simulink model "Simscape_Drone_Model"  (R2025b)
settings: Solver=FixedStepAuto  StartTime=0.0  StopTime=10  RelTol=1e-6  EnableMultiTasking=on
undefined symbols (not defined in the file): Aero_On, Config, P, SimParams, SimscapeParams, X, Y, Z
libraries: sm_lib x89, nesl_utility x71, fl_lib x18, sdl_lib x8, slpidlib x4, batteryecm_lib x1
(part 4 of 5)

== system Simscape_Drone_Model/Drone Mechanical/Motor Holder 1 ==
  rho : Inport
  Motor Holder 1 : sm_lib/Body Elements/Cylindrical Solid  CylinderRadius=SimscapeParams.MotorRadius  CylinderRadiusUnits=m  CylinderLength=SimscapeParams.MotorHeight  CylinderLengthUnits=m  ExportEntireGeometry=off  InertiaType=CalculateFromGeometry  BasedOnType=Mass  Density=1000  DensityUnits=kg/m^3  Mass=SimscapeParams.MotorMass  MassUnits=kg  CenterOfMass=[0 0 0]  CenterOfMassUnits=m  MomentsOfInertia=[1 1 1]  MomentsOfInertiaUnits=kg*m^2  ProductsOfInertia=[0 0 0]  ProductsOfInertiaUnits=kg*m^2  GraphicType=FromGeometry  MarkerShape=Sphere  MarkerSize=10  GraphicVisPropType=SimpleVisualProperties  GraphicDiffuseColor=[0.898 1 0]  GraphicOpacity=1  GraphicSpecularColor=[0.5 0.5 0.5 1.0]  GraphicAmbientColor=[0.15 0.15 0.15 1.0]  GraphicEmissiveColor=[0.0 0.0 0.0 1.0]  GraphicShininess=75  DoExposeReferenceFrame=off  SerializedFrames=|
      | <Frames>
      | 
      |   <Frame>
      |     <Id>Frame1</Id>
      |     <Value>
      |       <Name>Top</Name>
      |       <Origin>
      |         <Source>GeometricFeature</Source>
      |         <FeatureName>bottom surface</FeatureName>
      |       </Origin>
      |       <PrimaryAxis>
      |         <DefinedDirection>+Z</DefinedDirection>
      |         <Source>ReferenceFrame</Source>
      |         <SourceDirection>+Z</SourceDirection>
      |         <FeatureName></FeatureName>
      |       </PrimaryAxis>
      |       <SecondaryAxis>
      |         <DefinedDirection>+X</DefinedDirection>
      |         <Source>ReferenceFrame</Source>
      |         <SourceDirection>+X</SourceDirection>
      |         <FeatureName></FeatureName>
      |       </SecondaryAxis>
      |     </Value>
      |   </Frame>
      | 
      |   <Frame>
      |     <Id>Frame2</Id>
      |     <Value>
      |       <Name>Side</Name>
      |       <Origin>
      |         <Source>GeometricFeature</Source>
      |         <FeatureName>side surface</FeatureName>
      |       </Origin>
      |       <PrimaryAxis>
      |         <DefinedDirection>+Z</DefinedDirection>
      |         <Source>ReferenceFrame</Source>
      |         <SourceDirection>+Z</SourceDirection>
      |         <FeatureName></FeatureName>
      |       </PrimaryAxis>
      |       <SecondaryAxis>
      |         <DefinedDirection>+X</DefinedDirection>
      |         <Source>ReferenceFrame</Source>
      |         <SourceDirection>-X</SourceDirection>
      |         <FeatureName></FeatureName>
      |       </SecondaryAxis>
      |     </Value>
      |   </Frame>
      | 
      | </Frames>
  Rigid Transform : sm_lib/Frames and Transforms/Rigid Transform  RotationMethod=ArbitraryAxis  FollAlignAxisA=+X  BaseAlignAxisA=+Y  FollAlignAxisB=+Y  BaseAlignAxisB=+Z  RotationStandardAxis=+Z  RotationAngle=SimscapeParams.MotorHolderRotationAngle  RotationAngleUnits=deg  RotationArbitraryAxis=SimscapeParams.MotorHolderRotationAxis1  RotationSequenceAxes=FollowerAxes  RotationSequence=YXY  RotationSequenceAngles=[0 90 0]  RotationSequenceAnglesUnits=deg  RotationMatrix=[1 0 0;0 1 0;0 0 1]  Quaternion=[1 0 0 0]  TranslationMethod=None  TranslationCartesianOffset=[0 0 0]  TranslationCartesianOffsetUnits=m  TranslationStandardAxis=+Z  TranslationStandardOffset=0  TranslationStandardOffsetUnits=m  TranslationROffset=0  TranslationROffsetUnits=m  TranslationThetaOffset=0  TranslationThetaOffsetUnits=deg  TranslationZOffset=0  TranslationZOffsetUnits=m
  Subsystem : Subsystem
  NED : PMIOPort  Side=Left
  Connection : PMIOPort  Port=2  Side=Left
  Side : PMIOPort  Port=3  Side=Left
  Propeller : PMIOPort  Port=4  Side=Right
  wires:
  rho/1 -> Subsystem/1(rho)
  connections:
  Rigid Transform/LConn1 -- Connection/RConn1
  Motor Holder 1/LConn1 -- Propeller/RConn1
  Rigid Transform/RConn1 -- Motor Holder 1/RConn1 -- Subsystem/RConn2 -- Subsystem/RConn1 -- Side/RConn1
  NED/RConn1 -- Subsystem/LConn1

== system Simscape_Drone_Model/Drone Mechanical/Motor Holder 2 ==
  rho : Inport
  Aero Dynamic Drag : Subsystem
  External Force and Torque : sm_lib/Forces and Torques/External Force and Torque  EnableForceX=off  EnableForceY=off  EnableForceZ=off  EnableForce=on  ForceResolutionFrame=AttachedFrame  EnableTorqueX=off  EnableTorqueY=off  EnableTorqueZ=off  EnableTorque=off  TorqueResolutionFrame=AttachedFrame
  Motor Holder 2 : sm_lib/Body Elements/Cylindrical Solid  CylinderRadius=SimscapeParams.MotorRadius  CylinderRadiusUnits=m  CylinderLength=SimscapeParams.MotorHeight  CylinderLengthUnits=m  ExportEntireGeometry=off  InertiaType=CalculateFromGeometry  BasedOnType=Mass  Density=1000  DensityUnits=kg/m^3  Mass=SimscapeParams.MotorMass  MassUnits=kg  CenterOfMass=[0 0 0]  CenterOfMassUnits=m  MomentsOfInertia=[1 1 1]  MomentsOfInertiaUnits=kg*m^2  ProductsOfInertia=[0 0 0]  ProductsOfInertiaUnits=kg*m^2  GraphicType=FromGeometry  MarkerShape=Sphere  MarkerSize=10  GraphicVisPropType=SimpleVisualProperties  GraphicDiffuseColor=[0.898 1 0]  GraphicOpacity=1  GraphicSpecularColor=[0.5 0.5 0.5 1.0]  GraphicAmbientColor=[0.15 0.15 0.15 1.0]  GraphicEmissiveColor=[0.0 0.0 0.0 1.0]  GraphicShininess=75  DoExposeReferenceFrame=off  SerializedFrames=|
      | <Frames>
      | 
      |   <Frame>
      |     <Id>Frame1</Id>
      |     <Value>
      |       <Name>Top</Name>
      |       <Origin>
      |         <Source>GeometricFeature</Source>
      |         <FeatureName>bottom surface</FeatureName>
      |       </Origin>
      |       <PrimaryAxis>
      |         <DefinedDirection>+Z</DefinedDirection>
      |         <Source>ReferenceFrame</Source>
      |         <SourceDirection>+Z</SourceDirection>
      |         <FeatureName></FeatureName>
      |       </PrimaryAxis>
      |       <SecondaryAxis>
      |         <DefinedDirection>+X</DefinedDirection>
      |         <Source>ReferenceFrame</Source>
      |         <SourceDirection>+X</SourceDirection>
      |         <FeatureName></FeatureName>
      |       </SecondaryAxis>
      |     </Value>
      |   </Frame>
      | 
      |   <Frame>
      |     <Id>Frame2</Id>
      |     <Value>
      |       <Name>Side</Name>
      |       <Origin>
      |         <Source>GeometricFeature</Source>
      |         <FeatureName>side surface</FeatureName>
      |       </Origin>
      |       <PrimaryAxis>
      |         <DefinedDirection>+Z</DefinedDirection>
      |         <Source>ReferenceFrame</Source>
      |         <SourceDirection>+Z</SourceDirection>
      |         <FeatureName></FeatureName>
      |       </PrimaryAxis>
      |       <SecondaryAxis>
      |         <DefinedDirection>+X</DefinedDirection>
      |         <Source>ReferenceFrame</Source>
      |         <SourceDirection>-X</SourceDirection>
      |         <FeatureName></FeatureName>
      |       </SecondaryAxis>
      |     </Value>
      |   </Frame>
      | 
      | </Frames>
  Rigid Transform : sm_lib/Frames and Transforms/Rigid Transform  RotationMethod=ArbitraryAxis  FollAlignAxisA=+X  BaseAlignAxisA=+Y  FollAlignAxisB=+Y  BaseAlignAxisB=+Z  RotationStandardAxis=+Z  RotationAngle=SimscapeParams.MotorHolderRotationAngle  RotationAngleUnits=deg  RotationArbitraryAxis=SimscapeParams.MotorHolderRotationAxis2  RotationSequenceAxes=BaseAxes  RotationSequence=XYX  RotationSequenceAngles=[0 90 0]  RotationSequenceAnglesUnits=deg  RotationMatrix=[1 0 0;0 1 0;0 0 1]  Quaternion=[1 0 0 0]  TranslationMethod=None  TranslationCartesianOffset=[0 0 0]  TranslationCartesianOffsetUnits=m  TranslationStandardAxis=+Z  TranslationStandardOffset=0  TranslationStandardOffsetUnits=m  TranslationROffset=0  TranslationROffsetUnits=m  TranslationThetaOffset=0  TranslationThetaOffsetUnits=deg  TranslationZOffset=0  TranslationZOffsetUnits=m
  Simulink-PS Converter : nesl_utility/Simulink-PS Converter  PhysicalDomain=network_engine_domain  SubClassName=ps_input  LeftPortType=input  RightPortType=output  PseudoPeriodic=off  Frequencies=[]  NoiseDistribution=none  NoiseParameters=[]  Unit=1  AffineConversion=off  FilteringAndDerivatives=provide  SimscapeFilterOrder=1  InputFilterTimeConstant=0.001  UdotUserProvided=0
  NED : PMIOPort  Side=Left
  Connection : PMIOPort  Port=2  Side=Left
  Side : PMIOPort  Port=3  Side=Left
  Propeller : PMIOPort  Port=4  Side=Right
  wires:
  Aero Dynamic Drag/1(F_drag) -> Simulink-PS Converter/1
  rho/1 -> Aero Dynamic Drag/1(rho)
  connections:
  External Force and Torque/LConn1 -- Simulink-PS Converter/RConn1
  Aero Dynamic Drag/LConn1 -- NED/RConn1
  Rigid Transform/LConn1 -- Connection/RConn1
  Side/RConn1 -- Rigid Transform/RConn1 -- External Force and Torque/RConn1 -- Aero Dynamic Drag/LConn2 -- Motor Holder 2/RConn1
  Motor Holder 2/LConn1 -- Propeller/RConn1

== system Simscape_Drone_Model/Drone Mechanical/Motor Holder 3 ==
  rho : Inport
  Aero Dynamic Drag : Subsystem
  External Force and Torque : sm_lib/Forces and Torques/External Force and Torque  EnableForceX=off  EnableForceY=off  EnableForceZ=off  EnableForce=on  ForceResolutionFrame=AttachedFrame  EnableTorqueX=off  EnableTorqueY=off  EnableTorqueZ=off  EnableTorque=off  TorqueResolutionFrame=AttachedFrame
  Motor Holder 3 : sm_lib/Body Elements/Cylindrical Solid  CylinderRadius=SimscapeParams.MotorRadius  CylinderRadiusUnits=m  CylinderLength=SimscapeParams.MotorHeight  CylinderLengthUnits=m  ExportEntireGeometry=off  InertiaType=CalculateFromGeometry  BasedOnType=Mass  Density=1000  DensityUnits=kg/m^3  Mass=SimscapeParams.MotorMass  MassUnits=kg  CenterOfMass=[0 0 0]  CenterOfMassUnits=m  MomentsOfInertia=[1 1 1]  MomentsOfInertiaUnits=kg*m^2  ProductsOfInertia=[0 0 0]  ProductsOfInertiaUnits=kg*m^2  GraphicType=FromGeometry  MarkerShape=Sphere  MarkerSize=10  GraphicVisPropType=SimpleVisualProperties  GraphicDiffuseColor=[0.898 1 0]  GraphicOpacity=1  GraphicSpecularColor=[0.5 0.5 0.5 1.0]  GraphicAmbientColor=[0.15 0.15 0.15 1.0]  GraphicEmissiveColor=[0.0 0.0 0.0 1.0]  GraphicShininess=75  DoExposeReferenceFrame=off  SerializedFrames=|
      | <Frames>
      | 
      |   <Frame>
      |     <Id>Frame1</Id>
      |     <Value>
      |       <Name>Top</Name>
      |       <Origin>
      |         <Source>GeometricFeature</Source>
      |         <FeatureName>bottom surface</FeatureName>
      |       </Origin>
      |       <PrimaryAxis>
      |         <DefinedDirection>+Z</DefinedDirection>
      |         <Source>ReferenceFrame</Source>
      |         <SourceDirection>+Z</SourceDirection>
      |         <FeatureName></FeatureName>
      |       </PrimaryAxis>
      |       <SecondaryAxis>
      |         <DefinedDirection>+X</DefinedDirection>
      |         <Source>ReferenceFrame</Source>
      |         <SourceDirection>+X</SourceDirection>
      |         <FeatureName></FeatureName>
      |       </SecondaryAxis>
      |     </Value>
      |   </Frame>
      | 
      |   <Frame>
      |     <Id>Frame2</Id>
      |     <Value>
      |       <Name>Side</Name>
      |       <Origin>
      |         <Source>GeometricFeature</Source>
      |         <FeatureName>side surface</FeatureName>
      |       </Origin>
      |       <PrimaryAxis>
      |         <DefinedDirection>+Z</DefinedDirection>
      |         <Source>ReferenceFrame</Source>
      |         <SourceDirection>+Z</SourceDirection>
      |         <FeatureName></FeatureName>
      |       </PrimaryAxis>
      |       <SecondaryAxis>
      |         <DefinedDirection>+X</DefinedDirection>
      |         <Source>ReferenceFrame</Source>
      |         <SourceDirection>-X</SourceDirection>
      |         <FeatureName></FeatureName>
      |       </SecondaryAxis>
      |     </Value>
      |   </Frame>
      | 
      | </Frames>
  Rigid Transform : sm_lib/Frames and Transforms/Rigid Transform  RotationMethod=ArbitraryAxis  FollAlignAxisA=+X  BaseAlignAxisA=+Y  FollAlignAxisB=+Y  BaseAlignAxisB=+Z  RotationStandardAxis=+Z  RotationAngle=SimscapeParams.MotorHolderRotationAngle  RotationAngleUnits=deg  RotationArbitraryAxis=SimscapeParams.MotorHolderRotationAxis3  RotationSequenceAxes=FollowerAxes  RotationSequence=YXY  RotationSequenceAngles=[0 90 0]  RotationSequenceAnglesUnits=deg  RotationMatrix=[1 0 0;0 1 0;0 0 1]  Quaternion=[1 0 0 0]  TranslationMethod=None  TranslationCartesianOffset=[0 0 0]  TranslationCartesianOffsetUnits=m  TranslationStandardAxis=+Z  TranslationStandardOffset=0  TranslationStandardOffsetUnits=m  TranslationROffset=0  TranslationROffsetUnits=m  TranslationThetaOffset=0  TranslationThetaOffsetUnits=deg  TranslationZOffset=0  TranslationZOffsetUnits=m
  Simulink-PS Converter : nesl_utility/Simulink-PS Converter  PhysicalDomain=network_engine_domain  SubClassName=ps_input  LeftPortType=input  RightPortType=output  PseudoPeriodic=off  Frequencies=[]  NoiseDistribution=none  NoiseParameters=[]  Unit=1  AffineConversion=off  FilteringAndDerivatives=provide  SimscapeFilterOrder=1  InputFilterTimeConstant=0.001  UdotUserProvided=0
  NED : PMIOPort  Side=Left
  Connection : PMIOPort  Port=2  Side=Left
  Propeller : PMIOPort  Port=3  Side=Right
  Side : PMIOPort  Port=4  Side=Right
  wires:
  rho/1 -> Aero Dynamic Drag/1(rho)
  Aero Dynamic Drag/1(F_drag) -> Simulink-PS Converter/1
  connections:
  Aero Dynamic Drag/LConn1 -- NED/RConn1
  External Force and Torque/LConn1 -- Simulink-PS Converter/RConn1
  Rigid Transform/LConn1 -- Connection/RConn1
  Rigid Transform/RConn1 -- Motor Holder 3/RConn1 -- Side/RConn1 -- Aero Dynamic Drag/LConn2 -- External Force and Torque/RConn1
  Propeller/RConn1 -- Motor Holder 3/LConn1

== system Simscape_Drone_Model/Drone Mechanical/Motor Holder 4 ==
  rho : Inport
  Aero Dynamic Drag : Subsystem
  External Force and Torque : sm_lib/Forces and Torques/External Force and Torque  EnableForceX=off  EnableForceY=off  EnableForceZ=off  EnableForce=on  ForceResolutionFrame=AttachedFrame  EnableTorqueX=off  EnableTorqueY=off  EnableTorqueZ=off  EnableTorque=off  TorqueResolutionFrame=AttachedFrame
  Motor Holder 4 : sm_lib/Body Elements/Cylindrical Solid  CylinderRadius=SimscapeParams.MotorRadius  CylinderRadiusUnits=m  CylinderLength=SimscapeParams.MotorHeight  CylinderLengthUnits=m  ExportEntireGeometry=off  InertiaType=CalculateFromGeometry  BasedOnType=Mass  Density=1000  DensityUnits=kg/m^3  Mass=SimscapeParams.MotorMass  MassUnits=kg  CenterOfMass=[0 0 0]  CenterOfMassUnits=m  MomentsOfInertia=[1 1 1]  MomentsOfInertiaUnits=kg*m^2  ProductsOfInertia=[0 0 0]  ProductsOfInertiaUnits=kg*m^2  GraphicType=FromGeometry  MarkerShape=Sphere  MarkerSize=10  GraphicVisPropType=SimpleVisualProperties  GraphicDiffuseColor=[0.898 1 0]  GraphicOpacity=1  GraphicSpecularColor=[0.5 0.5 0.5 1.0]  GraphicAmbientColor=[0.15 0.15 0.15 1.0]  GraphicEmissiveColor=[0.0 0.0 0.0 1.0]  GraphicShininess=75  DoExposeReferenceFrame=off  SerializedFrames=|
      | <Frames>
      | 
      |   <Frame>
      |     <Id>Frame1</Id>
      |     <Value>
      |       <Name>Top</Name>
      |       <Origin>
      |         <Source>GeometricFeature</Source>
      |         <FeatureName>bottom surface</FeatureName>
      |       </Origin>
      |       <PrimaryAxis>
      |         <DefinedDirection>+Z</DefinedDirection>
      |         <Source>ReferenceFrame</Source>
      |         <SourceDirection>+Z</SourceDirection>
      |         <FeatureName></FeatureName>
      |       </PrimaryAxis>
      |       <SecondaryAxis>
      |         <DefinedDirection>+X</DefinedDirection>
      |         <Source>ReferenceFrame</Source>
      |         <SourceDirection>+X</SourceDirection>
      |         <FeatureName></FeatureName>
      |       </SecondaryAxis>
      |     </Value>
      |   </Frame>
      | 
      |   <Frame>
      |     <Id>Frame2</Id>
      |     <Value>
      |       <Name>Side</Name>
      |       <Origin>
      |         <Source>GeometricFeature</Source>
      |         <FeatureName>side surface</FeatureName>
      |       </Origin>
      |       <PrimaryAxis>
      |         <DefinedDirection>+Z</DefinedDirection>
      |         <Source>ReferenceFrame</Source>
      |         <SourceDirection>+Z</SourceDirection>
      |         <FeatureName></FeatureName>
      |       </PrimaryAxis>
      |       <SecondaryAxis>
      |         <DefinedDirection>+X</DefinedDirection>
      |         <Source>ReferenceFrame</Source>
      |         <SourceDirection>-X</SourceDirection>
      |         <FeatureName></FeatureName>
      |       </SecondaryAxis>
      |     </Value>
      |   </Frame>
      | 
      | </Frames>
  Rigid Transform : sm_lib/Frames and Transforms/Rigid Transform  RotationMethod=ArbitraryAxis  FollAlignAxisA=+X  BaseAlignAxisA=+Y  FollAlignAxisB=+Y  BaseAlignAxisB=+Z  RotationStandardAxis=+Z  RotationAngle=SimscapeParams.MotorHolderRotationAngle  RotationAngleUnits=deg  RotationArbitraryAxis=SimscapeParams.MotorHolderRotationAxis4  RotationSequenceAxes=FollowerAxes  RotationSequence=YXY  RotationSequenceAngles=[0 90 0]  RotationSequenceAnglesUnits=deg  RotationMatrix=[1 0 0;0 1 0;0 0 1]  Quaternion=[1 0 0 0]  TranslationMethod=None  TranslationCartesianOffset=[0 0 0]  TranslationCartesianOffsetUnits=m  TranslationStandardAxis=+Z  TranslationStandardOffset=0  TranslationStandardOffsetUnits=m  TranslationROffset=0  TranslationROffsetUnits=m  TranslationThetaOffset=0  TranslationThetaOffsetUnits=deg  TranslationZOffset=0  TranslationZOffsetUnits=m
  Simulink-PS Converter : nesl_utility/Simulink-PS Converter  PhysicalDomain=network_engine_domain  SubClassName=ps_input  LeftPortType=input  RightPortType=output  PseudoPeriodic=off  Frequencies=[]  NoiseDistribution=none  NoiseParameters=[]  Unit=1  AffineConversion=off  FilteringAndDerivatives=provide  SimscapeFilterOrder=1  InputFilterTimeConstant=0.001  UdotUserProvided=0
  NED : PMIOPort  Side=Left
  Connection : PMIOPort  Port=2  Side=Left
  Propeller : PMIOPort  Port=3  Side=Right
  Side : PMIOPort  Port=4  Side=Right
  wires:
  rho/1 -> Aero Dynamic Drag/1(rho)
  Aero Dynamic Drag/1(F_drag) -> Simulink-PS Converter/1
  connections:
  Aero Dynamic Drag/LConn1 -- NED/RConn1
  External Force and Torque/LConn1 -- Simulink-PS Converter/RConn1
  Rigid Transform/LConn1 -- Connection/RConn1
  Rigid Transform/RConn1 -- Side/RConn1 -- Motor Holder 4/RConn1 -- External Force and Torque/RConn1 -- Aero Dynamic Drag/LConn2
  Motor Holder 4/LConn1 -- Propeller/RConn1

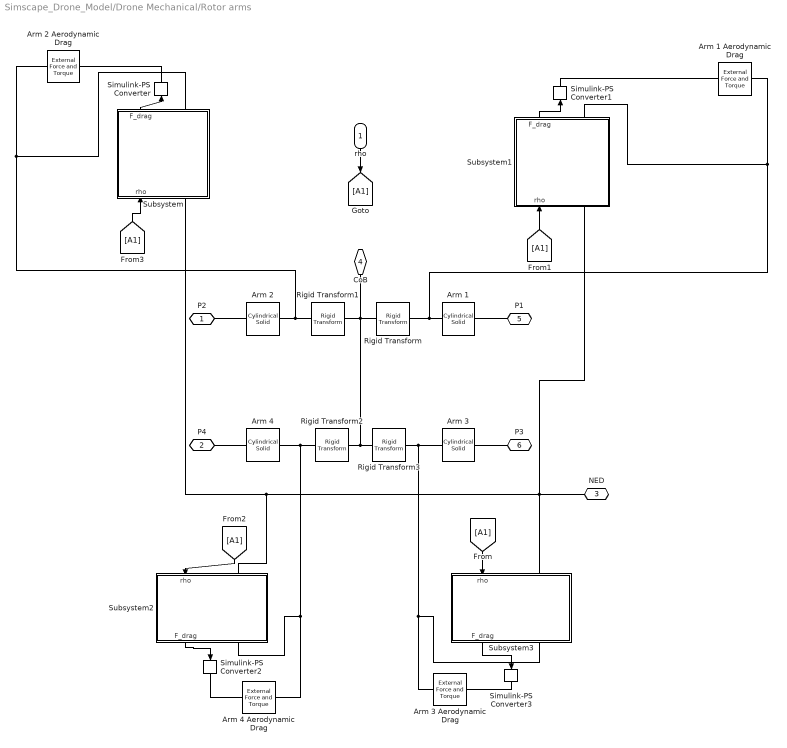
== system Simscape_Drone_Model/Drone Mechanical/Rotor arms ==
  rho : Inport
  Arm 1 : sm_lib/Body Elements/Cylindrical Solid  CylinderRadius=SimscapeParams.ArmRadius  CylinderRadiusUnits=m  CylinderLength=SimscapeParams.ArmLength  CylinderLengthUnits=m  ExportEntireGeometry=off  InertiaType=CalculateFromGeometry  BasedOnType=Mass  Density=1000  DensityUnits=kg/m^3  Mass=SimscapeParams.ArmMass  MassUnits=kg  CenterOfMass=[0 0 0]  CenterOfMassUnits=m  MomentsOfInertia=[1 1 1]  MomentsOfInertiaUnits=kg*m^2  ProductsOfInertia=[0 0 0]  ProductsOfInertiaUnits=kg*m^2  GraphicType=FromGeometry  MarkerShape=Sphere  MarkerSize=10  GraphicVisPropType=SimpleVisualProperties  GraphicDiffuseColor=[0 0.702 1]  GraphicOpacity=1  GraphicSpecularColor=[0.5 0.5 0.5 1.0]  GraphicAmbientColor=[0.15 0.15 0.15 1.0]  GraphicEmissiveColor=[0.0 0.0 0.0 1.0]  GraphicShininess=75  DoExposeReferenceFrame=on  SerializedFrames=|
      | <Frames>
      | 
      |   <Frame>
      |     <Id>Frame1</Id>
      |     <Value>
      |       <Name>F2</Name>
      |       <Origin>
      |         <Source>GeometricFeature</Source>
      |         <FeatureName>top surface</FeatureName>
      |       </Origin>
      |       <PrimaryAxis>
      |         <DefinedDirection>+Z</DefinedDirection>
      |         <Source>ReferenceFrame</Source>
      |         <SourceDirection>+Z</SourceDirection>
      |         <FeatureName></FeatureName>
      |       </PrimaryAxis>
      |       <SecondaryAxis>
      |         <DefinedDirection>+X</DefinedDirection>
      |         <Source>ReferenceFrame</Source>
      |         <SourceDirection>+X</SourceDirection>
      |         <FeatureName></FeatureName>
      |       </SecondaryAxis>
      |     </Value>
      |   </Frame>
      | 
      | </Frames>
  Arm 1 Aerodynamic Drag : sm_lib/Forces and Torques/External Force and Torque  EnableForceX=off  EnableForceY=off  EnableForceZ=off  EnableForce=on  ForceResolutionFrame=AttachedFrame  EnableTorqueX=off  EnableTorqueY=off  EnableTorqueZ=off  EnableTorque=off  TorqueResolutionFrame=AttachedFrame
  Arm 2 : sm_lib/Body Elements/Cylindrical Solid  CylinderRadius=SimscapeParams.ArmRadius  CylinderRadiusUnits=m  CylinderLength=SimscapeParams.ArmLength  CylinderLengthUnits=m  ExportEntireGeometry=off  InertiaType=CalculateFromGeometry  BasedOnType=Mass  Density=1000  DensityUnits=kg/m^3  Mass=SimscapeParams.ArmMass  MassUnits=kg  CenterOfMass=[0 0 0]  CenterOfMassUnits=m  MomentsOfInertia=[1 1 1]  MomentsOfInertiaUnits=kg*m^2  ProductsOfInertia=[0 0 0]  ProductsOfInertiaUnits=kg*m^2  GraphicType=FromGeometry  MarkerShape=Sphere  MarkerSize=10  GraphicVisPropType=SimpleVisualProperties  GraphicDiffuseColor=[0 0.702 1]  GraphicOpacity=1  GraphicSpecularColor=[0.5 0.5 0.5 1.0]  GraphicAmbientColor=[0.15 0.15 0.15 1.0]  GraphicEmissiveColor=[0.0 0.0 0.0 1.0]  GraphicShininess=75  DoExposeReferenceFrame=on  SerializedFrames=|
      | <Frames>
      | 
      |   <Frame>
      |     <Id>Frame1</Id>
      |     <Value>
      |       <Name>F2</Name>
      |       <Origin>
      |         <Source>GeometricFeature</Source>
      |         <FeatureName>top surface</FeatureName>
      |       </Origin>
      |       <PrimaryAxis>
      |         <DefinedDirection>+Z</DefinedDirection>
      |         <Source>ReferenceFrame</Source>
      |         <SourceDirection>+Z</SourceDirection>
      |         <FeatureName></FeatureName>
      |       </PrimaryAxis>
      |       <SecondaryAxis>
      |         <DefinedDirection>+X</DefinedDirection>
      |         <Source>ReferenceFrame</Source>
      |         <SourceDirection>+X</SourceDirection>
      |         <FeatureName></FeatureName>
      |       </SecondaryAxis>
      |     </Value>
      |   </Frame>
      | 
      | </Frames>
  Arm 2 Aerodynamic Drag : sm_lib/Forces and Torques/External Force and Torque  EnableForceX=off  EnableForceY=off  EnableForceZ=off  EnableForce=on  ForceResolutionFrame=AttachedFrame  EnableTorqueX=off  EnableTorqueY=off  EnableTorqueZ=off  EnableTorque=off  TorqueResolutionFrame=AttachedFrame
  Arm 3 : sm_lib/Body Elements/Cylindrical Solid  CylinderRadius=SimscapeParams.ArmRadius  CylinderRadiusUnits=m  CylinderLength=SimscapeParams.ArmLength  CylinderLengthUnits=m  ExportEntireGeometry=off  InertiaType=CalculateFromGeometry  BasedOnType=Mass  Density=1000  DensityUnits=kg/m^3  Mass=SimscapeParams.ArmMass  MassUnits=kg  CenterOfMass=[0 0 0]  CenterOfMassUnits=m  MomentsOfInertia=[1 1 1]  MomentsOfInertiaUnits=kg*m^2  ProductsOfInertia=[0 0 0]  ProductsOfInertiaUnits=kg*m^2  GraphicType=FromGeometry  MarkerShape=Sphere  MarkerSize=10  GraphicVisPropType=SimpleVisualProperties  GraphicDiffuseColor=[0 0.702 1]  GraphicOpacity=1  GraphicSpecularColor=[0.5 0.5 0.5 1.0]  GraphicAmbientColor=[0.15 0.15 0.15 1.0]  GraphicEmissiveColor=[0.0 0.0 0.0 1.0]  GraphicShininess=75  DoExposeReferenceFrame=on  SerializedFrames=|
      | <Frames>
      | 
      |   <Frame>
      |     <Id>Frame1</Id>
      |     <Value>
      |       <Name>F2</Name>
      |       <Origin>
      |         <Source>GeometricFeature</Source>
      |         <FeatureName>top surface</FeatureName>
      |       </Origin>
      |       <PrimaryAxis>
      |         <DefinedDirection>+Z</DefinedDirection>
      |         <Source>ReferenceFrame</Source>
      |         <SourceDirection>+Z</SourceDirection>
      |         <FeatureName></FeatureName>
      |       </PrimaryAxis>
      |       <SecondaryAxis>
      |         <DefinedDirection>+X</DefinedDirection>
      |         <Source>ReferenceFrame</Source>
      |         <SourceDirection>+X</SourceDirection>
      |         <FeatureName></FeatureName>
      |       </SecondaryAxis>
      |     </Value>
      |   </Frame>
      | 
      | </Frames>
  Arm 3 Aerodynamic Drag : sm_lib/Forces and Torques/External Force and Torque  EnableForceX=off  EnableForceY=off  EnableForceZ=off  EnableForce=on  ForceResolutionFrame=AttachedFrame  EnableTorqueX=off  EnableTorqueY=off  EnableTorqueZ=off  EnableTorque=off  TorqueResolutionFrame=AttachedFrame
  Arm 4 : sm_lib/Body Elements/Cylindrical Solid  CylinderRadius=SimscapeParams.ArmRadius  CylinderRadiusUnits=m  CylinderLength=SimscapeParams.ArmLength  CylinderLengthUnits=m  ExportEntireGeometry=off  InertiaType=CalculateFromGeometry  BasedOnType=Mass  Density=1000  DensityUnits=kg/m^3  Mass=SimscapeParams.ArmMass  MassUnits=kg  CenterOfMass=[0 0 0]  CenterOfMassUnits=m  MomentsOfInertia=[1 1 1]  MomentsOfInertiaUnits=kg*m^2  ProductsOfInertia=[0 0 0]  ProductsOfInertiaUnits=kg*m^2  GraphicType=FromGeometry  MarkerShape=Sphere  MarkerSize=10  GraphicVisPropType=SimpleVisualProperties  GraphicDiffuseColor=[0 0.702 1]  GraphicOpacity=1  GraphicSpecularColor=[0.5 0.5 0.5 1.0]  GraphicAmbientColor=[0.15 0.15 0.15 1.0]  GraphicEmissiveColor=[0.0 0.0 0.0 1.0]  GraphicShininess=75  DoExposeReferenceFrame=on  SerializedFrames=|
      | <Frames>
      | 
      |   <Frame>
      |     <Id>Frame1</Id>
      |     <Value>
      |       <Name>F2</Name>
      |       <Origin>
      |         <Source>GeometricFeature</Source>
      |         <FeatureName>top surface</FeatureName>
      |       </Origin>
      |       <PrimaryAxis>
      |         <DefinedDirection>+Z</DefinedDirection>
      |         <Source>ReferenceFrame</Source>
      |         <SourceDirection>+Z</SourceDirection>
      |         <FeatureName></FeatureName>
      |       </PrimaryAxis>
      |       <SecondaryAxis>
      |         <DefinedDirection>+X</DefinedDirection>
      |         <Source>ReferenceFrame</Source>
      |         <SourceDirection>+X</SourceDirection>
      |         <FeatureName></FeatureName>
      |       </SecondaryAxis>
      |     </Value>
      |   </Frame>
      | 
      | </Frames>
  Arm 4 Aerodynamic Drag : sm_lib/Forces and Torques/External Force and Torque  EnableForceX=off  EnableForceY=off  EnableForceZ=off  EnableForce=on  ForceResolutionFrame=AttachedFrame  EnableTorqueX=off  EnableTorqueY=off  EnableTorqueZ=off  EnableTorque=off  TorqueResolutionFrame=AttachedFrame
  Rigid Transform : sm_lib/Frames and Transforms/Rigid Transform  RotationMethod=ArbitraryAxis  FollAlignAxisA=+X  BaseAlignAxisA=+Y  FollAlignAxisB=+Y  BaseAlignAxisB=+Z  RotationStandardAxis=+Z  RotationAngle=SimscapeParams.ArmRotationAngle  RotationAngleUnits=deg  RotationArbitraryAxis=SimscapeParams.ArmRotationAxis1  RotationSequenceAxes=FollowerAxes  RotationSequence=XYZ  RotationSequenceAngles=P.Arm.RotationAngle.*P.Arm.RotationAxis1  RotationSequenceAnglesUnits=deg  RotationMatrix=[1 0 0;0 1 0;0 0 1]  Quaternion=[1 0 0 0]  TranslationMethod=Cartesian  TranslationCartesianOffset=SimscapeParams.ArmPosition1  TranslationCartesianOffsetUnits=m  TranslationStandardAxis=+Z  TranslationStandardOffset=0  TranslationStandardOffsetUnits=m  TranslationROffset=0  TranslationROffsetUnits=m  TranslationThetaOffset=0  TranslationThetaOffsetUnits=deg  TranslationZOffset=0  TranslationZOffsetUnits=m
  Rigid Transform1 : sm_lib/Frames and Transforms/Rigid Transform  RotationMethod=ArbitraryAxis  FollAlignAxisA=+X  BaseAlignAxisA=+Y  FollAlignAxisB=+Y  BaseAlignAxisB=+Z  RotationStandardAxis=+Z  RotationAngle=SimscapeParams.ArmRotationAngle  RotationAngleUnits=deg  RotationArbitraryAxis=SimscapeParams.ArmRotationAxis2  RotationSequenceAxes=FollowerAxes  RotationSequence=XYZ  RotationSequenceAngles=[-90 -45 0]  RotationSequenceAnglesUnits=deg  RotationMatrix=[1 0 0;0 1 0;0 0 1]  Quaternion=[1 0 0 0]  TranslationMethod=Cartesian  TranslationCartesianOffset=SimscapeParams.ArmPosition2  TranslationCartesianOffsetUnits=m  TranslationStandardAxis=+Z  TranslationStandardOffset=0  TranslationStandardOffsetUnits=m  TranslationROffset=0  TranslationROffsetUnits=m  TranslationThetaOffset=0  TranslationThetaOffsetUnits=deg  TranslationZOffset=0  TranslationZOffsetUnits=m
  Rigid Transform2 : sm_lib/Frames and Transforms/Rigid Transform  RotationMethod=ArbitraryAxis  FollAlignAxisA=+X  BaseAlignAxisA=+Y  FollAlignAxisB=+Y  BaseAlignAxisB=+Z  RotationStandardAxis=+Z  RotationAngle=SimscapeParams.ArmRotationAngle  RotationAngleUnits=deg  RotationArbitraryAxis=SimscapeParams.ArmRotationAxis4  RotationSequenceAxes=FollowerAxes  RotationSequence=XYZ  RotationSequenceAngles=[-90 -45 0]  RotationSequenceAnglesUnits=deg  RotationMatrix=[1 0 0;0 1 0;0 0 1]  Quaternion=[1 0 0 0]  TranslationMethod=Cartesian  TranslationCartesianOffset=SimscapeParams.ArmPosition4  TranslationCartesianOffsetUnits=m  TranslationStandardAxis=+Z  TranslationStandardOffset=0  TranslationStandardOffsetUnits=m  TranslationROffset=0  TranslationROffsetUnits=m  TranslationThetaOffset=0  TranslationThetaOffsetUnits=deg  TranslationZOffset=0  TranslationZOffsetUnits=m
  Rigid Transform3 : sm_lib/Frames and Transforms/Rigid Transform  RotationMethod=ArbitraryAxis  FollAlignAxisA=+X  BaseAlignAxisA=+Y  FollAlignAxisB=+Y  BaseAlignAxisB=+Z  RotationStandardAxis=+Z  RotationAngle=SimscapeParams.ArmRotationAngle  RotationAngleUnits=deg  RotationArbitraryAxis=SimscapeParams.ArmRotationAxis3  RotationSequenceAxes=FollowerAxes  RotationSequence=XYZ  RotationSequenceAngles=[-90 -45 0]  RotationSequenceAnglesUnits=deg  RotationMatrix=[1 0 0;0 1 0;0 0 1]  Quaternion=[1 0 0 0]  TranslationMethod=Cartesian  TranslationCartesianOffset=SimscapeParams.ArmPosition3  TranslationCartesianOffsetUnits=m  TranslationStandardAxis=+Z  TranslationStandardOffset=0  TranslationStandardOffsetUnits=m  TranslationROffset=0  TranslationROffsetUnits=m  TranslationThetaOffset=0  TranslationThetaOffsetUnits=deg  TranslationZOffset=0  TranslationZOffsetUnits=m
  Simulink-PS Converter{,1..3} (4 alike) : nesl_utility/Simulink-PS Converter  PhysicalDomain=network_engine_domain  SubClassName=ps_input  LeftPortType=input  RightPortType=output  PseudoPeriodic=off  Frequencies=[]  NoiseDistribution=none  NoiseParameters=[]  Unit=1  AffineConversion=off  FilteringAndDerivatives=provide  SimscapeFilterOrder=1  InputFilterTimeConstant=0.001  UdotUserProvided=0
  Subsystem : Subsystem
  Subsystem1 : Subsystem
  Subsystem2 : Subsystem
  Subsystem3 : Subsystem
  P2 : PMIOPort  Side=Left
  P4 : PMIOPort  Port=2  Side=Left
  NED : PMIOPort  Port=3  Side=Left
  CoB : PMIOPort  Port=4  Side=Left
  P1 : PMIOPort  Port=5  Side=Right
  P3 : PMIOPort  Port=6  Side=Right
  wires:
  rho/1 -> [A1]
  [A1] -> Subsystem/1(rho)
  Subsystem/1(F_drag) -> Simulink-PS Converter/1
  [A1] -> Subsystem1/1(rho)
  Subsystem1/1(F_drag) -> Simulink-PS Converter1/1
  [A1] -> Subsystem2/1(rho)
  Subsystem2/1(F_drag) -> Simulink-PS Converter2/1
  [A1] -> Subsystem3/1(rho)
  Subsystem3/1(F_drag) -> Simulink-PS Converter3/1
  connections:
  Arm 3 Aerodynamic Drag/LConn1 -- Simulink-PS Converter3/RConn1
  Arm 4 Aerodynamic Drag/LConn1 -- Simulink-PS Converter2/RConn1
  P2/RConn1 -- Arm 2/LConn1
  Arm 4/LConn1 -- P4/RConn1
  Arm 3/LConn1 -- P3/RConn1
  Arm 1/LConn1 -- P1/RConn1
  Rigid Transform3/RConn1 -- Arm 3/RConn1 -- Subsystem3/RConn1 -- Arm 3 Aerodynamic Drag/RConn1
  Arm 1 Aerodynamic Drag/LConn1 -- Simulink-PS Converter1/RConn1
  Arm 2 Aerodynamic Drag/LConn1 -- Simulink-PS Converter/RConn1
  Arm 2/RConn1 -- Rigid Transform1/RConn1 -- Subsystem/RConn1 -- Arm 2 Aerodynamic Drag/RConn1
  Arm 1/RConn1 -- Rigid Transform/RConn1 -- Subsystem1/RConn1 -- Arm 1 Aerodynamic Drag/RConn1
  Rigid Transform1/LConn1 -- CoB/RConn1 -- Rigid Transform2/LConn1 -- Rigid Transform3/LConn1 -- Rigid Transform/LConn1
  Subsystem3/LConn1 -- Subsystem1/LConn1 -- NED/RConn1 -- Subsystem/LConn1 -- Subsystem2/LConn1
  Rigid Transform2/RConn1 -- Arm 4/RConn1 -- Arm 4 Aerodynamic Drag/RConn1 -- Subsystem2/RConn1

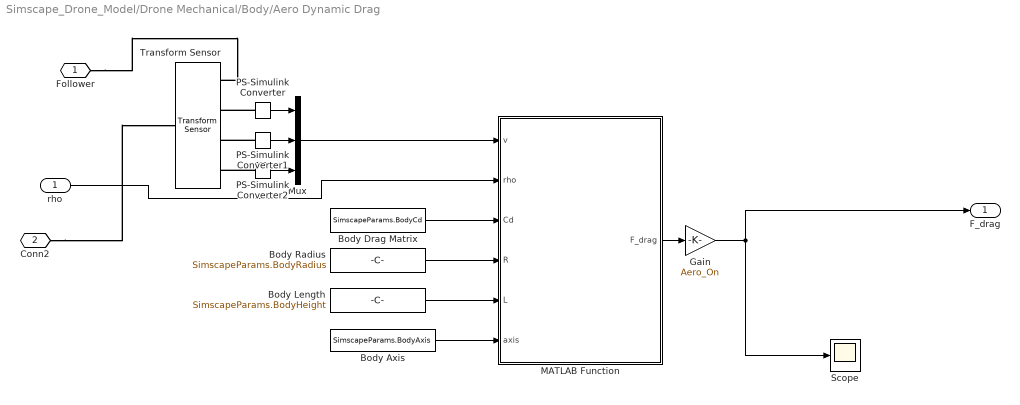
== system Simscape_Drone_Model/Drone Mechanical/Body/Aero Dynamic Drag ==
  rho : Inport
  Body Axis : Constant  Value=SimscapeParams.BodyAxis
  Body Drag Matrix : Constant  Value=SimscapeParams.BodyCd
  Body Length : Constant  Value=SimscapeParams.BodyHeight
  Body Radius : Constant  Value=SimscapeParams.BodyRadius
  Gain : Gain  Gain=Aero_On
  MATLAB Function : MATLAB Function  TreatAsAtomicUnit=on
  Mux : Mux  Inputs=3
  PS-Simulink Converter : nesl_utility/PS-Simulink Converter  PhysicalDomain=network_engine_domain  SubClassName=ps_output  LeftPortType=input  RightPortType=output  PseudoPeriodic=off  Frequencies=[]  VectorFormat=inherit  Unit=inherit  AffineConversion=off
  PS-Simulink Converter1 : nesl_utility/PS-Simulink Converter  PhysicalDomain=network_engine_domain  SubClassName=ps_output  LeftPortType=input  RightPortType=output  PseudoPeriodic=off  Frequencies=[]  VectorFormat=inherit  Unit=inherit  AffineConversion=off
  PS-Simulink Converter2 : nesl_utility/PS-Simulink Converter  PhysicalDomain=network_engine_domain  SubClassName=ps_output  LeftPortType=input  RightPortType=output  PseudoPeriodic=off  Frequencies=[]  VectorFormat=inherit  Unit=inherit  AffineConversion=off
  Scope : Scope
      settings: ActiveDisplayYMinimum=-1  ActiveDisplayYMaximum=1  DataLoggingVariableName=ScopeData4
  Transform Sensor : sm_lib/Frames and Transforms/Transform Sensor  MeasurementFrame=NonRotatingFollower  RotationSequence=XYZ  SenseAngle=off  SenseAxis=off  SenseQ=off  SenseR=off  SenseRotationSequence=off  SenseOmegaX=off  SenseOmegaY=off  SenseOmegaZ=off  SenseOmega=off  SenseQDot=off  SenseRDot=off  SenseRotationSequenceDot=off  SenseAlphaX=off  SenseAlphaY=off  SenseAlphaZ=off  SenseAlpha=off  SenseQDDot=off  SenseRDDot=off  SenseX=off  SenseY=off  SenseZ=off  SenseXYZ=off  SenseRad=off  SenseAzim=off  SenseDist=off  SenseInc=off  SenseXDot=on  SenseYDot=on  SenseZDot=on  SenseXYZDot=off  SenseRadDot=off  SenseAzimDot=off  SenseDistDot=off  SenseIncDot=off  SenseXDDot=off  SenseYDDot=off  SenseZDDot=off  SenseXYZDDot=off  SenseRadDDot=off  SenseAzimDDot=off  SenseDistDDot=off  SenseIncDDot=off
  Follower : PMIOPort  Side=Right
  Conn2 : PMIOPort  Port=2  Side=Left
  F_drag : Outport
  wires:
  Body Axis/1 -> MATLAB Function/6(axis)
  Body Drag Matrix/1 -> MATLAB Function/3(Cd)
  PS-Simulink Converter/1 -> Mux/1
  PS-Simulink Converter1/1 -> Mux/2
  Body Radius/1 -> MATLAB Function/4(R)
  Body Length/1 -> MATLAB Function/5(L)
  MATLAB Function/1(F_drag) -> Gain/1
  rho/1 -> MATLAB Function/2(rho)
  PS-Simulink Converter2/1 -> Mux/3
  Mux/1 -> MATLAB Function/1(v)
  Gain/1 -> F_drag/1, Scope/1
  connections:
  PS-Simulink Converter2/LConn1 -- Transform Sensor/RConn4
  PS-Simulink Converter1/LConn1 -- Transform Sensor/RConn3
  Conn2/RConn1 -- Transform Sensor/LConn1
  Follower/RConn1 -- Transform Sensor/RConn1
  PS-Simulink Converter/LConn1 -- Transform Sensor/RConn2

== system Simscape_Drone_Model/Drone Mechanical/Body/Collsioin ==
  PS-Simulink Converter : nesl_utility/PS-Simulink Converter  PhysicalDomain=network_engine_domain  SubClassName=ps_output  LeftPortType=input  RightPortType=output  PseudoPeriodic=off  Frequencies=[]  VectorFormat=inherit  Unit=inherit  AffineConversion=off
  PS-Simulink Converter1 : nesl_utility/PS-Simulink Converter  PhysicalDomain=network_engine_domain  SubClassName=ps_output  LeftPortType=input  RightPortType=output  PseudoPeriodic=off  Frequencies=[]  VectorFormat=inherit  Unit=inherit  AffineConversion=off
  PS-Simulink Converter2 : nesl_utility/PS-Simulink Converter  PhysicalDomain=network_engine_domain  SubClassName=ps_output  LeftPortType=input  RightPortType=output  PseudoPeriodic=off  Frequencies=[]  VectorFormat=inherit  Unit=inherit  AffineConversion=off
  Point Cloud : sm_lib/Curves and Surfaces/Point Cloud  CoordinatesMatrix=SimscapeParams.BodySurfacePoints  CoordinatesMatrixUnits=m  GraphicType=MarkerCloud  GraphicSphereRadius=1e-2  GraphicSphereRadiusUnits=m  GraphicVisPropType=SimpleVisualProperties  GraphicDiffuseColor=[0.5 0.5 0.5]  GraphicOpacity=1  GraphicSpecularColor=[0.5 0.5 0.5 1.0]  GraphicAmbientColor=[0.15 0.15 0.15 1.0]  GraphicEmissiveColor=[0.0 0.0 0.0 1.0]  GraphicShininess=75
  Scope : Scope  Commented=on  NumInputPorts=3
      settings: ActiveDisplayYMinimum=-0.12499999999999997  ActiveDisplayYMaximum=1.125  DataLoggingVariableName=ScopeData3
  Spatial Contact Force1 : sm_lib/Forces and Torques/Spatial Contact Force  SenseSeparationDistance=off  NormalForceType=SmoothSpringDamper  NormalStiffness=2.5e4  NormalStiffnessUnits=N/m  NormalDamping=50  NormalDampingUnits=N/(m/s)  NormalTransitionRegionWidth=1e-3  NormalTransitionRegionWidthUnits=m  FrictionType=None  CoefficientOfStaticFriction=0.8  CoefficientOfDynamicFriction=0.5  FrictionalCriticalVelocity=1e-2  FrictionalCriticalVelocityUnits=m/s  SenseContactSignal=on  SensePenetrationDepth=off  SenseNormalVelocity=off  SenseTangentialVelocity=on  SensingForceTorqueDirection=BaseOnFollower  SensingForceTorqueResolutionFrame=BaseFrame  SenseNormalForce=off  SenseNormalForceMagnitude=off  SenseNormalTorque=off  SenseFrictionalForce=on  SenseFrictionalForceMagnitude=off  SenseFrictionalTorque=off  SenseTotalForce=off  SenseTotalTorque=off  SenseContactBaseRotation=off  SenseContactBaseTranslation=off  SenseContactFollowerRotation=off  SenseContactFollowerTranslation=off  ZeroCrossDetectContactStartAndEnd=off
  Side : PMIOPort  Side=Left
  Body Collision : PMIOPort  Port=2  Side=Right
  wires:
  PS-Simulink Converter2/1 -> Scope/3  "Tangential Velocity"
  PS-Simulink Converter1/1 -> Scope/2  "Frictional Force"
  PS-Simulink Converter/1 -> Scope/1  "Contact"
  connections:
  PS-Simulink Converter2/LConn1 -- Spatial Contact Force1/RConn4
  PS-Simulink Converter1/LConn1 -- Spatial Contact Force1/RConn3
  PS-Simulink Converter/LConn1 -- Spatial Contact Force1/RConn2
  Side/RConn1 -- Point Cloud/LConn1
  Spatial Contact Force1/LConn1 -- Point Cloud/RConn1
  Spatial Contact Force1/RConn1 -- Body Collision/RConn1

== system Simscape_Drone_Model/Drone Mechanical/Body/Top Payload ==
  rho : Inport
  Top Payload : Subsystem  VariantControl=TopPayloadVariant == 1
      settings: PortSchema="{\"entries\":[{\"content\":{\"sides\":[{\"content\":{\"connectorIds\":[\"In1\",\"LConn1\",\"LConn2\"]},\"type\":\"ConnectorPlacement.EquallySpacedRectSide\",\"uuid\":\"c539331e-7ba0-423e-8576-0b8592caf2fb\"},{\"content\":{\"side\":\"RIGHT\"},\"type\":\"ConnectorPlacement.EquallySpacedRectSide\",\"uuid\":\"79846b77-3dcb-4e42-8a89-82d45755810a\"},{\"content\":{\"connectorIds\":[\"LConn3\"],\"side\":\"TOP\"},\"type\":\"ConnectorPlacement.EquallySpacedRectSide\",\"uuid\":\"7d0ca275-b432-428d-ad5e-1795dcc6a411\"}]},\"type\":\"ConnectorPlacement.EquallySpacedConnector\",\"uuid\":\"234f2347-aeac-4155-b9d7-055953fbd58b\"}],\"packageUris\":[\"http://schema.mathworks.com/mf0/Connector/R2020b\"],\"version\":\"1.0\"}"
  Top Connection : PMIOPort  Side=Left
  NED : PMIOPort  Port=2  Side=Left
  Body Collision : PMIOPort  Port=3  Side=Left

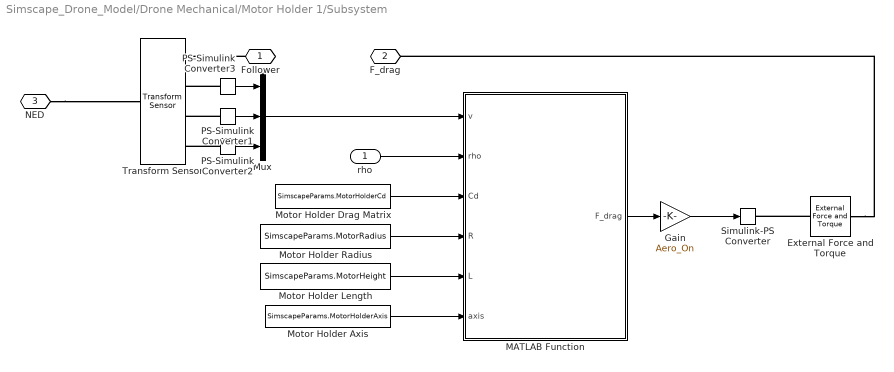
== system Simscape_Drone_Model/Drone Mechanical/Motor Holder 1/Subsystem ==
  rho : Inport
  External Force and Torque : sm_lib/Forces and Torques/External Force and Torque  EnableForceX=off  EnableForceY=off  EnableForceZ=off  EnableForce=on  ForceResolutionFrame=AttachedFrame  EnableTorqueX=off  EnableTorqueY=off  EnableTorqueZ=off  EnableTorque=off  TorqueResolutionFrame=AttachedFrame
  Gain : Gain  Gain=Aero_On
  MATLAB Function : MATLAB Function  TreatAsAtomicUnit=on
  Motor Holder Axis : Constant  Value=SimscapeParams.MotorHolderAxis
  Motor Holder Drag Matrix : Constant  Value=SimscapeParams.MotorHolderCd
  Motor Holder Length : Constant  Value=SimscapeParams.MotorHeight
  Motor Holder Radius : Constant  Value=SimscapeParams.MotorRadius
  Mux : Mux  Inputs=3
  PS-Simulink Converter1 : nesl_utility/PS-Simulink Converter  PhysicalDomain=network_engine_domain  SubClassName=ps_output  LeftPortType=input  RightPortType=output  PseudoPeriodic=off  Frequencies=[]  VectorFormat=inherit  Unit=inherit  AffineConversion=off
  PS-Simulink Converter2 : nesl_utility/PS-Simulink Converter  PhysicalDomain=network_engine_domain  SubClassName=ps_output  LeftPortType=input  RightPortType=output  PseudoPeriodic=off  Frequencies=[]  VectorFormat=inherit  Unit=inherit  AffineConversion=off
  PS-Simulink Converter3 : nesl_utility/PS-Simulink Converter  PhysicalDomain=network_engine_domain  SubClassName=ps_output  LeftPortType=input  RightPortType=output  PseudoPeriodic=off  Frequencies=[]  VectorFormat=inherit  Unit=inherit  AffineConversion=off
  Simulink-PS Converter : nesl_utility/Simulink-PS Converter  PhysicalDomain=network_engine_domain  SubClassName=ps_input  LeftPortType=input  RightPortType=output  PseudoPeriodic=off  Frequencies=[]  NoiseDistribution=none  NoiseParameters=[]  Unit=1  AffineConversion=off  FilteringAndDerivatives=provide  SimscapeFilterOrder=1  InputFilterTimeConstant=0.001  UdotUserProvided=0
  Transform Sensor : sm_lib/Frames and Transforms/Transform Sensor  MeasurementFrame=NonRotatingFollower  RotationSequence=XYZ  SenseAngle=off  SenseAxis=off  SenseQ=off  SenseR=off  SenseRotationSequence=off  SenseOmegaX=off  SenseOmegaY=off  SenseOmegaZ=off  SenseOmega=off  SenseQDot=off  SenseRDot=off  SenseRotationSequenceDot=off  SenseAlphaX=off  SenseAlphaY=off  SenseAlphaZ=off  SenseAlpha=off  SenseQDDot=off  SenseRDDot=off  SenseX=off  SenseY=off  SenseZ=off  SenseXYZ=off  SenseRad=off  SenseAzim=off  SenseDist=off  SenseInc=off  SenseXDot=on  SenseYDot=on  SenseZDot=on  SenseXYZDot=off  SenseRadDot=off  SenseAzimDot=off  SenseDistDot=off  SenseIncDot=off  SenseXDDot=off  SenseYDDot=off  SenseZDDot=off  SenseXYZDDot=off  SenseRadDDot=off  SenseAzimDDot=off  SenseDistDDot=off  SenseIncDDot=off
  Follower : PMIOPort  Side=Right
  F_drag : PMIOPort  Port=2  Side=Right
  NED : PMIOPort  Port=3  Side=Left
  wires:
  MATLAB Function/1(F_drag) -> Gain/1
  Mux/1 -> MATLAB Function/1(v)
  PS-Simulink Converter2/1 -> Mux/3
  PS-Simulink Converter3/1 -> Mux/1
  Motor Holder Length/1 -> MATLAB Function/5(L)
  Motor Holder Drag Matrix/1 -> MATLAB Function/3(Cd)
  PS-Simulink Converter1/1 -> Mux/2
  Motor Holder Radius/1 -> MATLAB Function/4(R)
  Motor Holder Axis/1 -> MATLAB Function/6(axis)
  rho/1 -> MATLAB Function/2(rho)
  Gain/1 -> Simulink-PS Converter/1
  connections:
  PS-Simulink Converter3/LConn1 -- Transform Sensor/RConn2
  External Force and Torque/LConn1 -- Simulink-PS Converter/RConn1
  External Force and Torque/RConn1 -- F_drag/RConn1
  PS-Simulink Converter1/LConn1 -- Transform Sensor/RConn3
  PS-Simulink Converter2/LConn1 -- Transform Sensor/RConn4
  NED/RConn1 -- Transform Sensor/LConn1
  Follower/RConn1 -- Transform Sensor/RConn1

== system Simscape_Drone_Model/Drone Mechanical/Motor Holder 2/Aero Dynamic Drag ==
  rho : Inport
  Gain : Gain  Gain=Aero_On
  MATLAB Function : MATLAB Function  TreatAsAtomicUnit=on
  Motor Holder Axis : Constant  Value=SimscapeParams.MotorHolderAxis
  Motor Holder Drag Matrix : Constant  Value=SimscapeParams.MotorHolderCd
  Motor Holder Length : Constant  Value=SimscapeParams.MotorHeight
  Motor Holder Radius : Constant  Value=SimscapeParams.MotorRadius
  Mux : Mux  Inputs=3
  PS-Simulink Converter : nesl_utility/PS-Simulink Converter  PhysicalDomain=network_engine_domain  SubClassName=ps_output  LeftPortType=input  RightPortType=output  PseudoPeriodic=off  Frequencies=[]  VectorFormat=inherit  Unit=inherit  AffineConversion=off
  PS-Simulink Converter1 : nesl_utility/PS-Simulink Converter  PhysicalDomain=network_engine_domain  SubClassName=ps_output  LeftPortType=input  RightPortType=output  PseudoPeriodic=off  Frequencies=[]  VectorFormat=inherit  Unit=inherit  AffineConversion=off
  PS-Simulink Converter2 : nesl_utility/PS-Simulink Converter  PhysicalDomain=network_engine_domain  SubClassName=ps_output  LeftPortType=input  RightPortType=output  PseudoPeriodic=off  Frequencies=[]  VectorFormat=inherit  Unit=inherit  AffineConversion=off
  Transform Sensor : sm_lib/Frames and Transforms/Transform Sensor  MeasurementFrame=NonRotatingFollower  RotationSequence=XYZ  SenseAngle=off  SenseAxis=off  SenseQ=off  SenseR=off  SenseRotationSequence=off  SenseOmegaX=off  SenseOmegaY=off  SenseOmegaZ=off  SenseOmega=off  SenseQDot=off  SenseRDot=off  SenseRotationSequenceDot=off  SenseAlphaX=off  SenseAlphaY=off  SenseAlphaZ=off  SenseAlpha=off  SenseQDDot=off  SenseRDDot=off  SenseX=off  SenseY=off  SenseZ=off  SenseXYZ=off  SenseRad=off  SenseAzim=off  SenseDist=off  SenseInc=off  SenseXDot=on  SenseYDot=on  SenseZDot=on  SenseXYZDot=off  SenseRadDot=off  SenseAzimDot=off  SenseDistDot=off  SenseIncDot=off  SenseXDDot=off  SenseYDDot=off  SenseZDDot=off  SenseXYZDDot=off  SenseRadDDot=off  SenseAzimDDot=off  SenseDistDDot=off  SenseIncDDot=off
  NED : PMIOPort  Side=Left
  F : PMIOPort  Port=2  Side=Left
  F_drag : Outport
  wires:
  PS-Simulink Converter/1 -> Mux/1
  PS-Simulink Converter2/1 -> Mux/3
  PS-Simulink Converter1/1 -> Mux/2
  rho/1 -> MATLAB Function/2(rho)
  Motor Holder Drag Matrix/1 -> MATLAB Function/3(Cd)
  Motor Holder Axis/1 -> MATLAB Function/6(axis)
  Motor Holder Radius/1 -> MATLAB Function/4(R)
  Motor Holder Length/1 -> MATLAB Function/5(L)
  Mux/1 -> MATLAB Function/1(v)
  MATLAB Function/1(F_drag) -> Gain/1
  Gain/1 -> F_drag/1
  connections:
  PS-Simulink Converter1/LConn1 -- Transform Sensor/RConn3
  PS-Simulink Converter2/LConn1 -- Transform Sensor/RConn4
  PS-Simulink Converter/LConn1 -- Transform Sensor/RConn2
  NED/RConn1 -- Transform Sensor/LConn1
  F/RConn1 -- Transform Sensor/RConn1

== system Simscape_Drone_Model/Drone Mechanical/Motor Holder 3/Aero Dynamic Drag ==
  rho : Inport
  Gain : Gain  Gain=Aero_On
  MATLAB Function : MATLAB Function  TreatAsAtomicUnit=on
  Motor Holder Axis : Constant  Value=SimscapeParams.MotorHolderAxis
  Motor Holder Drag Matrix : Constant  Value=SimscapeParams.MotorHolderCd
  Motor Holder Length : Constant  Value=SimscapeParams.MotorHeight
  Motor Holder Radius : Constant  Value=SimscapeParams.MotorRadius
  Mux : Mux  Inputs=3
  PS-Simulink Converter : nesl_utility/PS-Simulink Converter  PhysicalDomain=network_engine_domain  SubClassName=ps_output  LeftPortType=input  RightPortType=output  PseudoPeriodic=off  Frequencies=[]  VectorFormat=inherit  Unit=inherit  AffineConversion=off
  PS-Simulink Converter1 : nesl_utility/PS-Simulink Converter  PhysicalDomain=network_engine_domain  SubClassName=ps_output  LeftPortType=input  RightPortType=output  PseudoPeriodic=off  Frequencies=[]  VectorFormat=inherit  Unit=inherit  AffineConversion=off
  PS-Simulink Converter2 : nesl_utility/PS-Simulink Converter  PhysicalDomain=network_engine_domain  SubClassName=ps_output  LeftPortType=input  RightPortType=output  PseudoPeriodic=off  Frequencies=[]  VectorFormat=inherit  Unit=inherit  AffineConversion=off
  Transform Sensor : sm_lib/Frames and Transforms/Transform Sensor  MeasurementFrame=NonRotatingFollower  RotationSequence=XYZ  SenseAngle=off  SenseAxis=off  SenseQ=off  SenseR=off  SenseRotationSequence=off  SenseOmegaX=off  SenseOmegaY=off  SenseOmegaZ=off  SenseOmega=off  SenseQDot=off  SenseRDot=off  SenseRotationSequenceDot=off  SenseAlphaX=off  SenseAlphaY=off  SenseAlphaZ=off  SenseAlpha=off  SenseQDDot=off  SenseRDDot=off  SenseX=off  SenseY=off  SenseZ=off  SenseXYZ=off  SenseRad=off  SenseAzim=off  SenseDist=off  SenseInc=off  SenseXDot=on  SenseYDot=on  SenseZDot=on  SenseXYZDot=off  SenseRadDot=off  SenseAzimDot=off  SenseDistDot=off  SenseIncDot=off  SenseXDDot=off  SenseYDDot=off  SenseZDDot=off  SenseXYZDDot=off  SenseRadDDot=off  SenseAzimDDot=off  SenseDistDDot=off  SenseIncDDot=off
  NED : PMIOPort  Side=Left
  F : PMIOPort  Port=2  Side=Left
  F_drag : Outport
  wires:
  PS-Simulink Converter/1 -> Mux/1
  PS-Simulink Converter2/1 -> Mux/3
  PS-Simulink Converter1/1 -> Mux/2
  rho/1 -> MATLAB Function/2(rho)
  Motor Holder Drag Matrix/1 -> MATLAB Function/3(Cd)
  Motor Holder Axis/1 -> MATLAB Function/6(axis)
  Motor Holder Radius/1 -> MATLAB Function/4(R)
  Motor Holder Length/1 -> MATLAB Function/5(L)
  Mux/1 -> MATLAB Function/1(v)
  MATLAB Function/1(F_drag) -> Gain/1
  Gain/1 -> F_drag/1
  connections:
  PS-Simulink Converter1/LConn1 -- Transform Sensor/RConn3
  PS-Simulink Converter2/LConn1 -- Transform Sensor/RConn4
  PS-Simulink Converter/LConn1 -- Transform Sensor/RConn2
  NED/RConn1 -- Transform Sensor/LConn1
  F/RConn1 -- Transform Sensor/RConn1
